simulink model "PFM"  (R2024a)
settings: Solver=ode15s  StartTime=0.0  StopTime=0.5  FixedStep=1e-8  RelTol=1e-5
values from neighbouring files (symbols this model uses):
  Cd = 33e-6    (= 3.3e-05)    [Results.m]
  Co = 200e-6    (= 0.0002)    [Results.m]
  Cpv = 100e-6    (= 0.0001)    [Results.m]
  Cr = 3e-6    (= 3e-06)    [Results.m]
  I1 = data.I1(N)    [Results.m]
  I2 = data.I2(N)    [Results.m]
  I3 = data.I3(N)    [Results.m]
  IR1 = Irradiance1    [Results.m]
  IR2 = Irradiance2    [Results.m]
  IR3 = Irradiance3    [Results.m]
  Lm = 8e-6    (= 8e-06)    [Results.m]
  Lr = 1e-6    (= 1e-06)    [Results.m]
  N = 3.5    [Results.m]
  Pactual = [data.P1(N) data.P2(N) data.P3(N)]    [Results.m]
  Rleak = 1    [Results.m]
  T = data.Temperature(N)    [Results.m]
  Vactual = [data.VP1(N) data.VP2(N) data.VP3(N)]    [Results.m]
  Vout = 120    [Results.m]
libraries: spsDiodeLib x8, spsParallelRLCBranchLib x7, spsCurrentMeasurementLib x7, spsMosfetLib x5, spsSeriesRLCBranchLib x3, spsPVArrayLib x3, spsVoltageMeasurementLib x3, spsOnDelayLib x2, spsLinearTransformerLib x1, spsDCVoltageSourceLib x1, spspowerguiLib x1
settings Model: Creator=user  LastModifiedBy=Donald
settings OptimizationCC: ZeroExternalMemoryAtStartup=off  ZeroInternalMemoryAtStartup=off
settings SFSimCC: SimTargetLang=C++
settings RTWCC: Toolchain=Microsoft Visual C++ 2017 v15.0 | CMake/nmake (64-bit Windows)  BuildConfiguration=Release  TargetLang=C++
settings GRTTargetCC: TargetLangStandard=C++11 (ISO)  CodeInterfacePackaging=C++ class

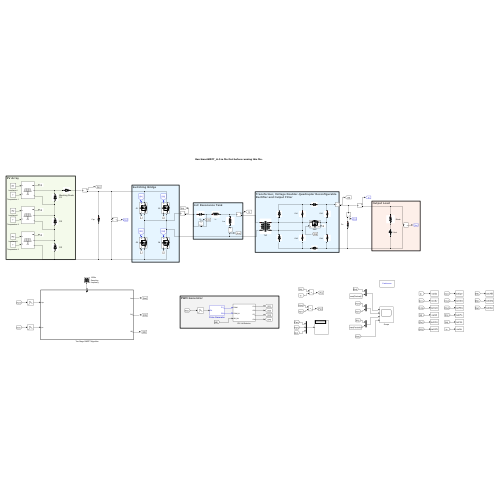
[thumbnail: Simulink's stored preview of the top-level diagram]
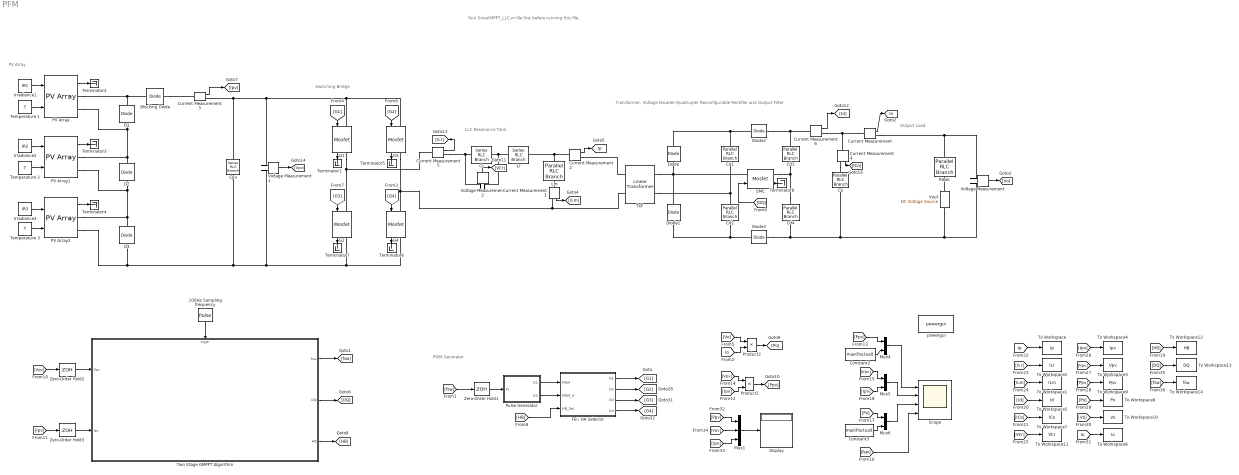
== system PFM ==
  note: LLC Resonance Tank
  note: PWM Generator
  note: PV Array
  note: Run SmartMPPT_LLC.m file first before running this file.
  note: Switching Bridge
  note: Output Load
  note: Transformer, Voltage Doubler-Quadrupler Reconfigurable
      | Rectifier and Output Filter
  100Hz Sampling frequency : DiscretePulseGenerator  PulseType=Time based  Period=1/100  PulseWidth=50
  Blocking Diode : spsDiodeLib/Diode  Ron=0.001  Lon=0  Vf=0.7  IC=0  UseSnubber=off  Rs=1e5*inf  Cs=inf  Measurements=off
  Cd{1..4} (4 alike) : spsParallelRLCBranchLib/Parallel RLC Branch  LConnTagsString=a  RConnTagsString=__new0  BranchType=C  Resistance=1  Inductance=1e-3  SetiL0=off  InitialCurrent=0  Capacitance=Cd  Setx0=off  InitialVoltage=0  Measurements=None
  Co : spsParallelRLCBranchLib/Parallel RLC Branch  LConnTagsString=a  RConnTagsString=__new0  BranchType=C  Resistance=1  Inductance=1e-3  SetiL0=off  InitialCurrent=0  Capacitance=Co  Setx0=off  InitialVoltage=0  Measurements=None
  Constant2 : Constant  Value=max(Pactual)
  Constant3 : Constant  Value=max(Pactual)
  Cpv : spsSeriesRLCBranchLib/Series RLC Branch  LConnTagsString=__new0  RConnTagsString=__new0  BranchType=C  Resistance=1  Inductance=1e-3  SetiL0=off  InitialCurrent=0  Capacitance=Cpv  Setx0=on  InitialVoltage=0  Measurements=None
  Cr : spsSeriesRLCBranchLib/Series RLC Branch  LConnTagsString=__new0  RConnTagsString=__new0  BranchType=C  Resistance=1  Inductance=1e-3  SetiL0=off  InitialCurrent=0  Capacitance=Cr  Setx0=off  InitialVoltage=0  Measurements=None
  Current Measurement{,1..6} (7 alike) : spsCurrentMeasurementLib/Current Measurement  PhasorSimulation=off  OutputType=Complex  PSBequivalent=0
  D1 : spsDiodeLib/Diode  Ron=0.001  Lon=0  Vf=0.7  IC=0  UseSnubber=off  Rs=1e5*inf  Cs=inf  Measurements=off
  D2 : spsDiodeLib/Diode  Ron=0.001  Lon=0  Vf=0.7  IC=0  UseSnubber=off  Rs=1e5*inf  Cs=inf  Measurements=off
  D3 : spsDiodeLib/Diode  Ron=0.001  Lon=0  Vf=0.7  IC=0  UseSnubber=off  Rs=1e5*inf  Cs=inf  Measurements=off
  Diode{,1..3} (4 alike) : spsDiodeLib/Diode  Ron=1e-3  Lon=0  Vf=0  IC=0  UseSnubber=0  Rs=inf  Cs=0  Measurements=off
  Display : Display
  FB / HA Selector : Subsystem
  G1 : spsMosfetLib/Mosfet  Ron=1e-3  Lon=0  Rd=1e-3  Vfd=0  IC=0  Rs=10e3  Cs=0.1e-6  Measurements=on
  G2 : spsMosfetLib/Mosfet  Ron=1e-3  Lon=0  Rd=1e-3  Vfd=0  IC=0  Rs=10e3  Cs=0.1e-6  Measurements=on
  G3 : spsMosfetLib/Mosfet  Ron=1e-3  Lon=0  Rd=1e-3  Vfd=0  IC=0  Rs=10e3  Cs=0  Measurements=on
  G4 : spsMosfetLib/Mosfet  Ron=1e-3  Lon=0  Rd=1e-3  Vfd=0  IC=0  Rs=10e3  Cs=0.1e-6  Measurements=on
  Irradiance1 : Constant  Value=IR1
  Irradiance2 : Constant  Value=IR2
  Irradiance3 : Constant  Value=IR3
  Lm : spsParallelRLCBranchLib/Parallel RLC Branch  LConnTagsString=a  RConnTagsString=__new0  BranchType=L  Resistance=1  Inductance=Lm  SetiL0=off  InitialCurrent=0  Capacitance=1e-6  Setx0=off  InitialVoltage=0  Measurements=None
  Lr : spsSeriesRLCBranchLib/Series RLC Branch  LConnTagsString=__new0  RConnTagsString=__new0  BranchType=L  Resistance=1  Inductance=Lr  SetiL0=off  InitialCurrent=0  Capacitance=2.91e-6  Setx0=off  InitialVoltage=0  Measurements=None
  Mux1 : Mux  Inputs=3
  Mux4 : Mux  Inputs=2
  Mux5 : Mux  Inputs=2
  Mux6 : Mux  Inputs=2
  PV Array : spsPVArrayLib/PV Array  Npar=1  Nser=1  PlotType=array @ 25 deg.C & specified irradiances  S_vec="[ 1000  600  100 ]"  Temp_C_vec="[ 45 25  ]"  ModuleName=User-defined  PlotWhenSelected=off  Pm=83.2824  Ncell=60/3  Voc=37.92*20/60  Isc=8.62  Vm=30.96*20/60  Im=8.07  beta_Voc_pc=-0.36099  alpha_Isc_pc=0.06371  beta_Voc=-0.045629  alpha_Isc=0.0054918  IL=8.6465  I0=3.0335e-10  nI=1.0227  Rsh=76.0432  Rs=0.09434  RobustModel=off  RobustCellTemperature=313.3991  BAL=on  Tc=1e-6  Tfilter=5e-5
  PV Array1 : spsPVArrayLib/PV Array  Npar=1  Nser=1  PlotType=array @ 25 deg.C & specified irradiances  S_vec="[ 1000  600  100 ]"  Temp_C_vec="[ 45 25  ]"  ModuleName=User-defined  PlotWhenSelected=off  Pm=83.2824  Ncell=60/3  Voc=37.92*20/60  Isc=8.62  Vm=30.96*20/60  Im=8.07  beta_Voc_pc=-0.36099  alpha_Isc_pc=0.06371  beta_Voc=-0.045629  alpha_Isc=0.0054918  IL=8.6465  I0=3.0335e-10  nI=1.0227  Rsh=76.0432  Rs=0.09434  RobustModel=off  RobustCellTemperature=313.3991  BAL=on  Tc=1e-6  Tfilter=5e-5
  PV Array2 : spsPVArrayLib/PV Array  Npar=1  Nser=1  PlotType=array @ 25 deg.C & specified irradiances  S_vec="[ 1000  600  100 ]"  Temp_C_vec="[ 45 25  ]"  ModuleName=User-defined  PlotWhenSelected=off  Pm=83.2824  Ncell=60/3  Voc=37.92*20/60  Isc=8.62  Vm=30.96*20/60  Im=8.07  beta_Voc_pc=-0.36099  alpha_Isc_pc=0.06371  beta_Voc=-0.045629  alpha_Isc=0.0054918  IL=8.6465  I0=3.0335e-10  nI=1.0227  Rsh=76.0432  Rs=0.09434  RobustModel=off  RobustCellTemperature=313.3991  BAL=on  Tc=1e-6  Tfilter=5e-5
  Product1 : Product
  Product2 : Product
  Pulse Generator : Subsystem
  Rleak : spsParallelRLCBranchLib/Parallel RLC Branch  LConnTagsString=a  RConnTagsString=__new0  BranchType=R  Resistance=Rleak  Inductance=1.193e-05  SetiL0=off  InitialCurrent=0  Capacitance=1e-6  Setx0=off  InitialVoltage=0  Measurements=None
  SMC : spsMosfetLib/Mosfet  Ron=1e-3  Lon=0  Rd=1e-3  Vfd=0  IC=0  Rs=10e3  Cs=0  Measurements=on
  Scope : Scope  NumInputPorts=4
  TXF : spsLinearTransformerLib/Linear Transformer  UNITS=pu  NominalPower=[1000 100e3 ]  winding1=[1 0 0]  winding2=[N 0 0]  ThreeWindings=off  winding3=[ 315e3 0.002 0.08 ]  RmLm=[ 1e6 inf ]  Measurements=None  DataType=off
  Temperature 1 : Constant  Value=T
  Temperature 2 : Constant  Value=T
  Temperature 3 : Constant  Value=T
  Terminator{1..8} (8 alike) : Terminator
  To Workspace : ToWorkspace  VariableName=Ip  SaveFormat=Timeseries  SampleTime=-1
  To Workspace1 : ToWorkspace  VariableName=ILm  SaveFormat=Timeseries  SampleTime=-1
  To Workspace10 : ToWorkspace  VariableName=Vo  SaveFormat=Timeseries  SampleTime=-1
  To Workspace11 : ToWorkspace  VariableName=VCr  SaveFormat=Timeseries  SampleTime=-1
  To Workspace12 : ToWorkspace  VariableName=HB  SaveFormat=Timeseries  SampleTime=-1
  To Workspace13 : ToWorkspace  VariableName=DQ  SaveFormat=Timeseries  SampleTime=-1
  To Workspace14 : ToWorkspace  VariableName=fsw  SaveFormat=Timeseries  SampleTime=-1
  To Workspace2 : ToWorkspace  VariableName=ILr  SaveFormat=Timeseries  SampleTime=-1
  To Workspace3 : ToWorkspace  VariableName=Vpv  SaveFormat=Timeseries  SampleTime=-1
  To Workspace4 : ToWorkspace  VariableName=Ipv  SaveFormat=Timeseries  SampleTime=-1
  To Workspace5 : ToWorkspace  VariableName=Id  SaveFormat=Timeseries  SampleTime=-1
  To Workspace6 : ToWorkspace  VariableName=Io  SaveFormat=Timeseries  SampleTime=-1
  To Workspace7 : ToWorkspace  VariableName=ICo  SaveFormat=Timeseries  SampleTime=-1
  To Workspace8 : ToWorkspace  VariableName=Po  SaveFormat=Timeseries  SampleTime=-1
  To Workspace9 : ToWorkspace  VariableName=Ppv  SaveFormat=Timeseries  SampleTime=-1
  Two Stage GMPPT Algorithm : Subsystem  TreatAsAtomicUnit=on
  Voltage Measurement : spsVoltageMeasurementLib/Voltage Measurement  PhasorSimulation=off  OutputType=Complex  PSBequivalent=0
  Voltage Measurement1 : spsVoltageMeasurementLib/Voltage Measurement  PhasorSimulation=off  OutputType=Complex  PSBequivalent=0
  Voltage Measurement2 : spsVoltageMeasurementLib/Voltage Measurement  PhasorSimulation=off  OutputType=Complex  PSBequivalent=0
  Vout : spsDCVoltageSourceLib/DC Voltage Source  Amplitude=Vout  Measurements=None
  Zero-Order Hold1 : ZeroOrderHold  SampleTime=1/100e3
  Zero-Order Hold2 : ZeroOrderHold  SampleTime=1/100e3
  Zero-Order Hold3 : ZeroOrderHold  SampleTime=1/100e3
  powergui : spspowerguiLib/powergui  Priority=1  SimulationMode=Continuous  SampleTime=1e-8  frequency=60  Iterations=50  frequencyindice=0  Pbase=100e6  ErrMax=1e-4  UnitsV=kV  UnitsW=MW  buscounter=0  FunctionMessages=off  echomessages=off  EnableUseOfTLC=off  CurrentSourceSwitches=off  DisableSnubberDevices=off  DisableRonSwitches=off  DisableVfSwitches=off  DisplayEquations=off  AutomaticDiscreteSolvers=off  SolverType=Tustin/Backward Euler (TBE)  Interpol=off  ExternalGateDelay=off  methode=off  Ts=100  x0status=blocks  SPID=on  SwTol=0  HookPort=off  NonlinearTolerance=1e-4  nMaxIteration=100  ContinueOnMaxIteration=off  RestoreLinks=warning  ResistiveCurrentMeasurement=off  Frange=[0:2:500]  Ylog=off  Xlog=on  ShowGrid=off  save=off  variable=ZData  structure=0  ZoomFFT=off  StartTime=0.0  cycles=1  DisplayStyle=1  fundamental=60  FreqAxis=off  MaxFrequency=1000  frequencyindicesteady=1  RmsSteady=1  display=off
  tag scope: Io=global, Ip=global
  wires:
  Current Measurement5/1 -> [ILr]
  Current Measurement1/1 -> [ILm]
  Current Measurement2/1 -> [Ip]
  [G4] -> G4/1
  [G1] -> G1/1
  [G3] -> G2/1
  [G2] -> G3/1
  Irradiance1/1 -> PV Array/1
  Irradiance2/1 -> PV Array1/1
  Irradiance3/1 -> PV Array2/1
  Temperature 2/1 -> PV Array1/2
  PV Array/1 -> Terminator2/1
  PV Array2/1 -> Terminator4/1
  Temperature 3/1 -> PV Array2/2
  PV Array1/1 -> Terminator3/1
  Temperature 1/1 -> PV Array/2
  Zero-Order Hold1/1 -> Pulse Generator/1(Fs)
  G1/1 -> Terminator1/1
  G3/1 -> Terminator5/1
  G4/1 -> Terminator6/1
  G2/1 -> Terminator7/1
  [DQ] -> SMC/1
  Current Measurement6/1 -> [Id]
  SMC/1 -> Terminator8/1
  Current Measurement4/1 -> [ICo]
  FB / HA Selector/3(G3) -> [G3]
  FB / HA Selector/2(G2) -> [G2]
  Pulse Generator/2(G2) -> FB / HA Selector/2(PWM_N)
  FB / HA Selector/4(G4) -> [G4]
  FB / HA Selector/1(G1) -> [G1]
  Pulse Generator/1(G1) -> FB / HA Selector/1(PWM)
  [fsw] -> Zero-Order Hold1/1
  100Hz Sampling frequency/1 -> Two Stage GMPPT Algorithm/Trigger
  Zero-Order Hold2/1 -> Two Stage GMPPT Algorithm/1(Vpv)
  Zero-Order Hold3/1 -> Two Stage GMPPT Algorithm/2(Ipv)
  Two Stage GMPPT Algorithm/1(fsw) -> [fsw]
  Two Stage GMPPT Algorithm/3(HB) -> [HB]
  Two Stage GMPPT Algorithm/2(DQ) -> [DQ]
  [HB] -> FB / HA Selector/3(HB_Sel)
  [Vpv] -> Zero-Order Hold2/1
  [Ipv] -> Zero-Order Hold3/1
  Current Measurement3/1 -> [Ipv]
  Voltage Measurement1/1 -> [Vpv]
  Voltage Measurement/1 -> [Vo]
  Current Measurement/1 -> [Io]
  Voltage Measurement2/1 -> [VCr]
  [Ppv] -> Mux1/1
  [Vo] -> To Workspace10/1
  [Po] -> To Workspace8/1
  [Ppv] -> To Workspace9/1
  [Vpv] -> To Workspace3/1
  [ICo] -> To Workspace7/1
  [Vo] -> Product2/1
  [Ipv] -> To Workspace4/1
  [Io] -> To Workspace6/1
  [Id] -> To Workspace5/1
  [VCr] -> To Workspace11/1
  [Ip] -> To Workspace/1
  [fsw] -> Scope/4
  Mux1/1 -> Display/1
  Product1/1 -> [Ppv]
  [Io] -> Product2/2
  Product2/1 -> [Po]
  [ILm] -> To Workspace1/1
  [Po] -> Mux6/1
  Constant2/1 -> Mux4/2
  Constant3/1 -> Mux6/2
  [Vpv] -> Product1/1
  Mux4/1 -> Scope/1
  [Ipv] -> Product1/2
  Mux6/1 -> Scope/3
  [Ipv] -> Mux1/3
  [Ipv] -> Mux5/2
  Mux5/1 -> Scope/2
  [Vpv] -> Mux1/2
  [Vpv] -> Mux5/1
  [ILr] -> To Workspace2/1
  [Ppv] -> Mux4/1
  [DQ] -> To Workspace13/1
  [HB] -> To Workspace12/1
  [fsw] -> To Workspace14/1
  connections:
  Lm/LConn1 -- Current Measurement2/LConn1 -- Lr/RConn1
  Lr/LConn1 -- Voltage Measurement2/LConn2 -- Cr/RConn1
  Voltage Measurement2/LConn1 -- Current Measurement5/RConn1 -- Cr/LConn1
  Lm/RConn1 -- Current Measurement1/LConn1
  TXF/LConn1 -- Current Measurement2/RConn1
  G3/RConn1 -- G4/LConn1 -- TXF/LConn2 -- Current Measurement1/RConn1
  G2/LConn1 -- G1/RConn1 -- Current Measurement5/LConn1
  G3/LConn1 -- Current Measurement3/RConn1 -- Cpv/LConn1 -- Voltage Measurement1/LConn1 -- G1/LConn1
  G2/RConn1 -- G4/RConn1 -- Voltage Measurement1/LConn2 -- Cpv/RConn1 -- D3/LConn1 -- PV Array2/RConn2
  PV Array1/RConn1 -- D2/RConn1 -- PV Array/RConn2 -- D1/LConn1
  PV Array1/RConn2 -- PV Array2/RConn1 -- D3/RConn1 -- D2/LConn1
  D1/RConn1 -- PV Array/RConn1 -- Blocking Diode/LConn1
  Blocking Diode/RConn1 -- Current Measurement3/LConn1
  Diode/RConn1 -- Diode2/LConn1 -- Cd1/LConn1
  Diode2/RConn1 -- Cd3/LConn1 -- Current Measurement6/LConn1
  Cd2/LConn1 -- TXF/RConn2 -- Cd1/RConn1
  Cd4/LConn1 -- Cd3/RConn1 -- SMC/RConn1
  Current Measurement/LConn1 -- Current Measurement4/LConn1 -- Current Measurement6/RConn1
  Diode1/RConn1 -- TXF/RConn1 -- SMC/LConn1 -- Diode/LConn1
  Voltage Measurement/LConn1 -- Rleak/LConn1 -- Current Measurement/RConn1
  Vout/LConn1 -- Voltage Measurement/LConn2 -- Co/RConn1 -- Cd4/RConn1 -- Diode3/LConn1
  Diode1/LConn1 -- Diode3/RConn1 -- Cd2/RConn1
  Vout/RConn1 -- Rleak/RConn1
  Current Measurement4/RConn1 -- Co/LConn1

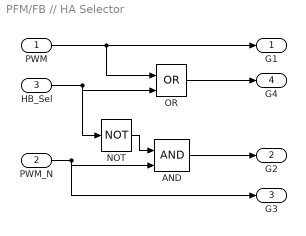
== system PFM/FB // HA Selector ==
  PWM : Inport
  PWM_N : Inport  Port=2
  HB_Sel : Inport  Port=3
  AND : Logic  IconShape=distinctive  AllPortsSameDT=off  OutDataTypeStr=boolean
  NOT : Logic  Operator=NOT  IconShape=distinctive  AllPortsSameDT=off  OutDataTypeStr=boolean
  OR : Logic  Operator=OR  IconShape=distinctive  AllPortsSameDT=off  OutDataTypeStr=boolean
  G1 : Outport
  G2 : Outport  Port=2
  G3 : Outport  Port=3
  G4 : Outport  Port=4
  wires:
  OR/1 -> G4/1
  PWM/1 -> OR/1, G1/1
  HB_Sel/1 -> NOT/1, OR/2
  PWM_N/1 -> AND/2, G3/1
  AND/1 -> G2/1
  NOT/1 -> AND/1

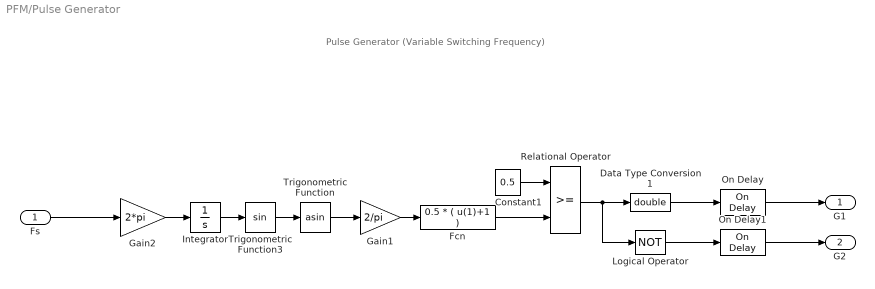
== system PFM/Pulse Generator ==
  note: Pulse Generator
      | (Variable Switching Frequency)
  Fs : Inport
  Constant1 : Constant  Value=0.5
  Data Type Conversion1 : DataTypeConversion  OutDataTypeStr=double  SaturateOnIntegerOverflow=off  RndMeth=Floor
  Fcn : Fcn  Expr=0.5 * ( u(1)+1 )
  Gain1 : Gain  Gain=2/pi  SaturateOnIntegerOverflow=on  OutDataTypeStr=Inherit: Same as input  ParamDataTypeStr=Inherit: Same as input
  Gain2 : Gain  Gain=2*pi  SaturateOnIntegerOverflow=on  OutDataTypeStr=Inherit: Same as input  ParamDataTypeStr=Inherit: Same as input
  Integrator : Integrator
  Logical Operator : Logic  Operator=NOT  AllPortsSameDT=off  OutDataTypeStr=float('double')
  On Delay : spsOnDelayLib/On Delay  DelayType=On delay  delay=400e-9  ic=0  Ts=0
  On Delay1 : spsOnDelayLib/On Delay  DelayType=On delay  delay=400e-9  ic=0  Ts=0
  Relational Operator : RelationalOperator  OutDataTypeStr=boolean  InputSameDT=off
  Trigonometric Function : Trigonometry  Operator=asin
  Trigonometric Function3 : Trigonometry
  G1 : Outport  VectorParamsAs1DForOutWhenUnconnected=off
  G2 : Outport  Port=2  VectorParamsAs1DForOutWhenUnconnected=off
  wires:
  Trigonometric Function3/1 -> Trigonometric Function/1
  Gain1/1 -> Fcn/1
  Trigonometric Function/1 -> Gain1/1
  Integrator/1 -> Trigonometric Function3/1
  Constant1/1 -> Relational Operator/1
  Relational Operator/1 -> Data Type Conversion1/1, Logical Operator/1
  Fcn/1 -> Relational Operator/2
  Logical Operator/1 -> On Delay1/1
  Data Type Conversion1/1 -> On Delay/1
  Gain2/1 -> Integrator/1
  Fs/1 -> Gain2/1
  On Delay/1 -> G1/1
  On Delay1/1 -> G2/1

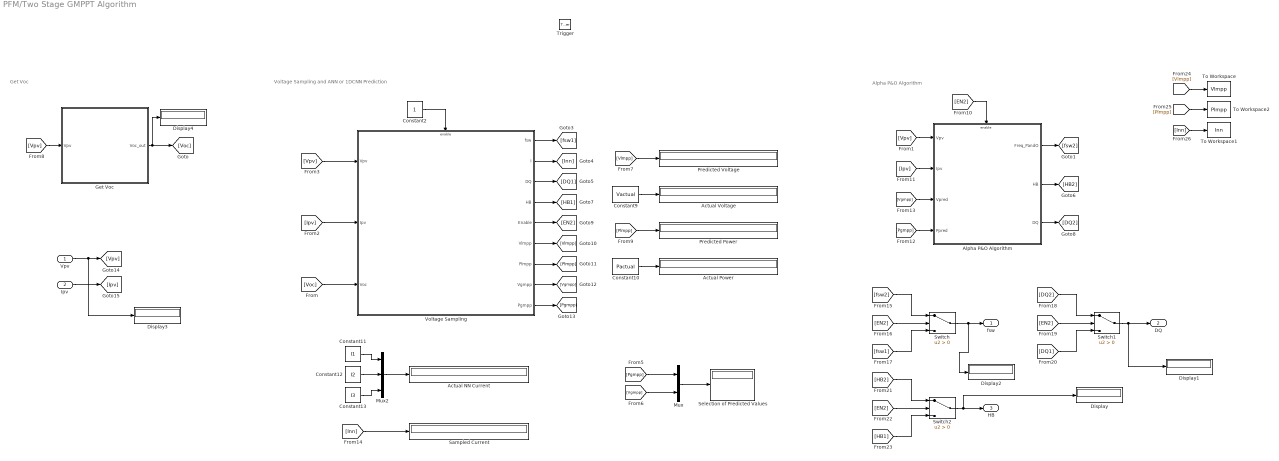
== system PFM/Two Stage GMPPT Algorithm ==
  note: Voltage Sampling and ANN or 1DCNN Prediction
  note: Alpha P&O Algorithm
  note: Get Voc
  Vpv : Inport
  Ipv : Inport  Port=2
  Trigger : TriggerPort  VariantControl=(inherit)  InitialTriggerSignalState=positive  PortDimensions=1
  Actual NN Current : Display
  Actual Power : Display
  Actual Voltage : Display
  Alpha P&O Algorithm : Subsystem  TreatAsAtomicUnit=on
  Constant10 : Constant  Value=Pactual
  Constant11 : Constant  Value=I1
  Constant12 : Constant  Value=I2
  Constant13 : Constant  Value=I3
  Constant2 : Constant
  Constant9 : Constant  Value=Vactual
  Display{,1..4} (5 alike) : Display
  Get Voc : MATLAB Function  TreatAsAtomicUnit=on
  Mux : Mux  Inputs=2
  Mux2 : Mux  Inputs=3
  Predicted Power : Display
  Predicted Voltage : Display
  Sampled Current : Display
  Selection of Predicted Values : Display
  Switch : Switch  Criteria=u2 > Threshold  SaturateOnIntegerOverflow=off  InputSameDT=off
  Switch1 : Switch  Criteria=u2 > Threshold  SaturateOnIntegerOverflow=off  InputSameDT=off
  Switch2 : Switch  Criteria=u2 > Threshold  SaturateOnIntegerOverflow=off  InputSameDT=off
  To Workspace : ToWorkspace  VariableName=Vlmpp  SaveFormat=Timeseries  SampleTime=-1
  To Workspace1 : ToWorkspace  VariableName=Inn  SaveFormat=Timeseries  SampleTime=-1
  To Workspace2 : ToWorkspace  VariableName=Plmpp  SaveFormat=Timeseries  SampleTime=-1
  Voltage Sampling : Subsystem  TreatAsAtomicUnit=on
  fsw : Outport
  DQ : Outport  Port=2
  HB : Outport  Port=3
  wires:
  Mux2/1 -> Actual NN Current/1
  [Pgmpp] -> Mux/1
  [EN2] -> Alpha P&O Algorithm/Enable
  Constant12/1 -> Mux2/2
  Alpha P&O Algorithm/1(Freq_PandO) -> [fsw2]
  Constant13/1 -> Mux2/3
  Constant11/1 -> Mux2/1
  Mux/1 -> Selection of Predicted Values/1
  [Voc] -> Voltage Sampling/3(Voc)
  [Vpv] -> Voltage Sampling/1(Vpv)
  [Ipv] -> Voltage Sampling/2(Ipv)
  Voltage Sampling/1(fsw) -> [fsw1]
  Voltage Sampling/2(I) -> [Inn]
  Voltage Sampling/9(Pgmpp) -> [Pgmpp]
  Voltage Sampling/8(Vgmpp) -> [Vgmpp]
  Voltage Sampling/7(Plmpp) -> [Plmpp]
  Voltage Sampling/6(Vlmpp) -> [Vlmpp]
  Voltage Sampling/5(Enable) -> [EN2]
  Voltage Sampling/4(HB) -> [HB1]
  Voltage Sampling/3(DQ) -> [DQ1]
  [Vgmpp] -> Mux/2
  Constant10/1 -> Actual Power/1
  [Plmpp] -> Predicted Power/1
  Constant9/1 -> Actual Voltage/1
  [Vlmpp] -> Predicted Voltage/1
  Alpha P&O Algorithm/2(HB) -> [HB2]
  Alpha P&O Algorithm/3(DQ) -> [DQ2]
  [Vpv] -> Alpha P&O Algorithm/1(Vpv)
  [Ipv] -> Alpha P&O Algorithm/2(Ipv)
  [Vgmpp] -> Alpha P&O Algorithm/3(Vpred)
  [Pgmpp] -> Alpha P&O Algorithm/4(Ppred)
  Vpv/1 -> Display3/1, [Vpv]
  Ipv/1 -> [Ipv]
  [Inn] -> Sampled Current/1
  [EN2] -> Switch/2
  [fsw2] -> Switch/1
  [fsw1] -> Switch/3
  Switch/1 -> Display2/1, fsw/1
  [DQ1] -> Switch1/3
  [DQ2] -> Switch1/1
  [EN2] -> Switch1/2
  Switch1/1 -> Display1/1, DQ/1
  Switch2/1 -> Display/1, HB/1
  [HB1] -> Switch2/3
  [HB2] -> Switch2/1
  [EN2] -> Switch2/2
  [Vpv] -> Get Voc/1(Vpv)
  Get Voc/1(Voc_out) -> [Voc], Display4/1
  Constant2/1 -> Voltage Sampling/Enable
  [Plmpp] -> To Workspace2/1
  [Inn] -> To Workspace1/1
  [Vlmpp] -> To Workspace/1

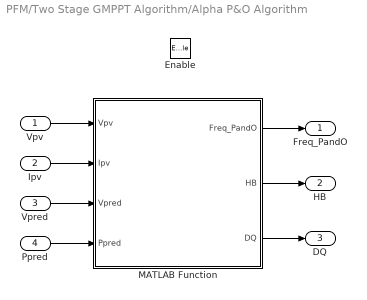
== system PFM/Two Stage GMPPT Algorithm/Alpha P&O Algorithm ==
  Vpv : Inport
  Ipv : Inport  Port=2
  Vpred : Inport  Port=3
  Ppred : Inport  Port=4
  Enable : EnablePort
  MATLAB Function : MATLAB Function  TreatAsAtomicUnit=on
  Freq_PandO : Outport
  HB : Outport  Port=2
  DQ : Outport  Port=3
  wires:
  Ppred/1 -> MATLAB Function/4(Ppred)
  Vpv/1 -> MATLAB Function/1(Vpv)
  MATLAB Function/3(DQ) -> DQ/1
  Vpred/1 -> MATLAB Function/3(Vpred)
  MATLAB Function/1(Freq_PandO) -> Freq_PandO/1
  MATLAB Function/2(HB) -> HB/1
  Ipv/1 -> MATLAB Function/2(Ipv)

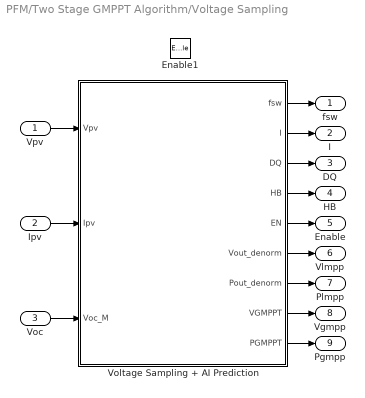
== system PFM/Two Stage GMPPT Algorithm/Voltage Sampling ==
  Vpv : Inport
  Ipv : Inport  Port=2
  Voc : Inport  Port=3
  Enable1 : EnablePort
  Voltage Sampling + AI Prediction : MATLAB Function  TreatAsAtomicUnit=on
  fsw : Outport
  I : Outport  Port=2
  DQ : Outport  Port=3
  HB : Outport  Port=4
  Enable : Outport  Port=5
  Vlmpp : Outport  Port=6
  Plmpp : Outport  Port=7
  Vgmpp : Outport  Port=8
  Pgmpp : Outport  Port=9
  wires:
  Voltage Sampling + AI Prediction/4(HB) -> HB/1
  Voltage Sampling + AI Prediction/3(DQ) -> DQ/1
  Voltage Sampling + AI Prediction/5(EN) -> Enable/1
  Voltage Sampling + AI Prediction/1(fsw) -> fsw/1
  Voltage Sampling + AI Prediction/2(I) -> I/1
  Vpv/1 -> Voltage Sampling + AI Prediction/1(Vpv)
  Ipv/1 -> Voltage Sampling + AI Prediction/2(Ipv)
  Voltage Sampling + AI Prediction/6(Vout_denorm) -> Vlmpp/1
  Voltage Sampling + AI Prediction/7(Pout_denorm) -> Plmpp/1
  Voltage Sampling + AI Prediction/8(VGMPPT) -> Vgmpp/1
  Voltage Sampling + AI Prediction/9(PGMPPT) -> Pgmpp/1
  Voc/1 -> Voltage Sampling + AI Prediction/3(Voc_M)

== matlab function PFM/Two Stage GMPPT Algorithm/Get Voc ==
  data: Vpv input; Voc_out output
function Voc_out  = VocSample(Vpv)
    % Store measurement for the current frequency.
    persistent Voc;
    
    % Initialize persistent variables only once
    if isempty(Voc)
        Voc = Vpv;
    end
    
    if Vpv > Voc
        Voc = Vpv;
    end
    Voc_out = Voc;
end

== matlab function PFM/Two Stage GMPPT Algorithm/Alpha P&O Algorithm/MATLAB Function ==
  data: Vpv input; Freq_PandO output; Ipv input; Vpred input; Ppred input; HB output; DQ output
function [Freq_PandO, HB, DQ] = PandO(Vpv, Ipv, Vpred, Ppred)
    % Constants.
    delta_freq = 2e3;
    
    % Current power.
    Ppv = Vpv * Ipv;
    
    % Persistent variables to retain values between function calls.
    persistent Vold Pold Fcalc HB_old DQ_old;

    % Initialize persistent variables on the first function call.
    if isempty(Fcalc)
        Vold = Vpred;        % Store the initial predicted voltage for ANN.
        Pold = Ppred;        % Store the initial predicted power for ANN.
        Fcalc = 0;
        if Vpred > 21
            DQ_old = 0;
            HB_old = 1;
            Gain = 120/Vpred /3.5/2*2;
            Fcalc = FMIM(Ppred, Gain);
        elseif Vpred > 11
            DQ_old = 0;
            HB_old = 0;
            Gain = 120/Vpred /3.5/2;
            Fcalc = FMIM(Ppred, Gain);
        else
            DQ_old = 1;
            HB_old = 0;
            Gain = 120/Vpred /3.5/2/2;
            Fcalc = FMIM(Ppred, Gain);
        end
        
        % Output initial voltage on the first call.
        Freq_PandO = Fcalc; 
        HB = HB_old;
        DQ = DQ_old;
        return;            % Exit early during initialization.
    end
    
    % Try use sigmoid.
    factor = 1/(1+exp(-abs(Ppv - Pold)));

    % P&O algorithm logic.
    if abs(Ppv - Pold) < 0.01  % Threshold to account for floating-point precision.
        % If power has not significantly changed, retain the previous
        % calculated frequency.
        Freq_PandO = Fcalc;
        HB = HB_old;
        DQ = DQ_old;
    else
        % Decide voltage adjustment based on power and voltage changes.
        if (Ppv - Pold) < 0
            % Power decreased
            if (Vpv - Vold) < 0
                Fcalc = Fcalc + delta_freq*factor; % Increase the voltage.
            else
                Fcalc = Fcalc - delta_freq*factor; % Decrease the voltage.
            end
        else
            % Power increased.
            if (Vpv - Vold) < 0
                Fcalc = Fcalc - delta_freq; % Decrease the voltage.
            else
                Fcalc = Fcalc + delta_freq; % Increase the voltage.
            end
        end
        
        % Update the output voltage after adjustment.
        Freq_PandO = Fcalc;
        HB = HB_old;
        DQ = DQ_old;
    end

    % Update the previous voltage and power for the next iteration.
    Vold = Vpv;
    Pold = Ppv;
end


function f0 = FMIM(P_assumed, Gain)
    % FMIM performs the initial switching frequency estimation based on
    % the FMIM method using an assumed power level.
    %
    % Inputs:
    %   Vref      - Reference voltage.
    %   P_assumed - Assumed power (W) (e.g., 50 or 100 W).
    %
    % Output:
    %   f0 - Estimated switching frequency.
    
    % LLC converter parameters.
    Cr = 3e-6;
    Lr = 1e-6;
    Lm = 8e-6;
    
    % Output voltage.
    Vout = 120;
    
    % Calculate load resistance assuming 100% efficiency.
    Rload = Vout^2 / P_assumed;
    % Transformer turns ratio.
    N = 1/5;
    % Effective AC resistance for full-bridge LLC converter.
    Rac = (8/pi^2) * (N^2) * (1/4) * Rload;
    
    % Define key parameters.
    K = Lm / Lr;
    Q = sqrt(Lr / Cr) / Rac;
    
    % Cubic equation's coefficients.
    a = 1;
    b = ((K^(-2)*(K+1)^2) - (2*Q^2) - (Gain^(-2))) / (Q^2);
    c = (Q^2 - (2*K^(-2) * (K + 1))) / (Q^2);
    d = (1 / (K * Q))^2;
    
    % Solve the cubic equation and take the square roots of the roots.
    fn_array = sqrt(roots([a b c d]));
    fn = max(real(fn_array));
    
    % Calculate resonance frequency.
    fr = 1 / (2 * pi * sqrt(Lr * Cr));
    
    % Estimated switching frequency.
    f0 = fn * fr;
end

== matlab function PFM/Two Stage GMPPT Algorithm/Voltage Sampling/Voltage Sampling + AI Prediction ==
  data: Vpv input; Ipv input; fsw output; I output; DQ output; HB output; EN output; Vout_denorm output; Pout_denorm output; VGMPPT output; PGMPPT output; Voc_M input
function [fsw, I, DQ, HB, EN, Vout_denorm, Pout_denorm, VGMPPT, PGMPPT] = SearchVref(Vpv, Ipv, Voc_M)
    % Store measurement for the current frequency.
    persistent NSample Vref targetVal Inn InnFlag fold DQ_Sel HB_EN ENC Vout_denorm_old Pout_denorm_old VGMPPT_old PGMPPT_old;
    
    if isempty(fold)
        % /////////////////////////////////////////////////////////////
        % Voltage scanning param.
        % /////////////////////////////////////////////////////////////
        NSample = 0;  
        Vref = [0.4*12.64, 0.4+12.64, 0.4+2*12.64];
        targetVal = Vref(1);
        Inn = zeros(1, 3);
        I = Inn;
        InnFlag = zeros(1,3);

        [fold, HB_EN, DQ_Sel] = initializeSearchVref(targetVal, 35);
        DQ = DQ_Sel;
        HB = HB_EN;

        % Copy frequency to persistence and 48kHz < fsw < 250kHz.
        fold = max(45e3, fold);
        fold = min(250e3, fold);
        fsw = fold;
        % /////////////////////////////////////////////////////////////
        
        % Done ANN and voltage sampling ?
        ENC = 0;
        EN = ENC;
        
        % ANN param.
        Vout_denorm_old = [0 0 0];
        Pout_denorm_old = [0 0 0];
        VGMPPT_old = 0;
        PGMPPT_old = 0;
        Vout_denorm = Vout_denorm_old;
        Pout_denorm = Pout_denorm_old;
        VGMPPT = VGMPPT_old;
        PGMPPT = PGMPPT_old;
        return;
    end
    
    
    if ENC == 0
        NSample = NSample + 1;
        
        % Check each target voltage (Threshold from Jerome).
        for i = 1:3
            if (abs(Vref(i) - Vpv) < 2.1) && ~InnFlag(i)
                Inn(i) = Ipv;
                InnFlag(i) = 1;
                if InnFlag(1) == 0
                    targetVal = Vref(1);
                    [fold, HB_EN, DQ_Sel] = initializeSearchVref(targetVal, 35);
                elseif InnFlag(2) == 0
                    targetVal = Vref(2);
                    [fold, HB_EN, DQ_Sel] = initializeSearchVref(targetVal, 70);
                elseif InnFlag(3) == 0
                    targetVal = Vref(3);
                    [fold, HB_EN, DQ_Sel] = initializeSearchVref(targetVal, 60);
                else
                    ENC = 1;
                    [Vout_denorm_old, Pout_denorm_old, VGMPPT_old, PGMPPT_old] = tflite_predict(double(Inn(1)), double(Inn(2)), double(Inn(3)), double(Voc_M));

                end
                DQ = DQ_Sel;
                HB = HB_EN;
                EN = ENC;
                fsw = fold;
                I = Inn;
                
                Vout_denorm = Vout_denorm_old;
                Pout_denorm = Pout_denorm_old;
                VGMPPT = VGMPPT_old;
                PGMPPT = PGMPPT_old;

                disp('--/////////////////////');
                disp(Vref);
                disp(Vpv);
                disp(fold);
                disp(Inn);
                disp(InnFlag);
                disp(NSample);
                disp('--/////////////////////');
                return;
            end
        end

        fold = sliding_surface_control(targetVal, Vpv, fold);
         
        % Constrain fsw to a valid range (40kHz to infinity Hz).
        fold = max(45e3, fold);
        fold = min(250e3, fold);
        
        DQ = DQ_Sel;
        HB = HB_EN;
        ENC = 0;
        EN = ENC;
        fsw = fold;
        I = Inn;
        
        Vout_denorm = Vout_denorm_old;
        Pout_denorm = Pout_denorm_old;
        VGMPPT = VGMPPT_old;
        PGMPPT = PGMPPT_old;

        disp('/////////////////////');
        disp(Vref);
        disp(Vpv);
        disp(fold);
        disp(Inn);
        disp(InnFlag);
        disp(NSample);
        disp('/////////////////////');
    else
        DQ = DQ_Sel;
        HB = HB_EN;
        EN = ENC;
        fsw = fold;
        I = Inn;

        Vout_denorm = Vout_denorm_old;
        Pout_denorm = Pout_denorm_old;
        VGMPPT = VGMPPT_old;
        PGMPPT = PGMPPT_old;
    end
end


function [fsw, HB, DQ] = initializeSearchVref(Vref, P)
        Pass = P;
        if Vref > 21
            DQ_Sel = 0;
            HB_EN = 1;
            Gain = 120/Vref /3.5/2*2;
            fold = FMIM(Pass, Gain);
        elseif Vref > 11
            DQ_Sel = 0;
            HB_EN = 0;
            Gain = 120/Vref /3.5/2;
            fold = FMIM(Pass, Gain);
        else
            DQ_Sel = 1;
            HB_EN = 0;
            Gain = 120/Vref /3.5/2/2;
            fold = FMIM(Pass, Gain);
        end
    
        % Copy frequency to persistence and 48kHz < fsw < 250kHz.
        fold = max(45e3, fold);
        fold = min(250e3, fold);
        fsw = fold;
        
        HB = HB_EN;
        DQ = DQ_Sel;
end


function f0 = FMIM(P_assumed, Gain)
    % FMIM performs the initial switching frequency estimation based on
    % the FMIM method using an assumed power level.
    %
    % Inputs:
    %   Vref      - Reference voltage.
    %   P_assumed - Assumed power (W) (e.g., 50 or 100 W).
    %
    % Output:
    %   f0 - Estimated switching frequency.
    
    % LLC converter parameters.
    Cr = 3e-6;
    Lr = 1e-6;
    Lm = 8e-6;
    
    % Output voltage.
    Vout = 120;
    
    % Calculate load resistance assuming 100% efficiency.
    Rload = Vout^2 / P_assumed;
    % Transformer turns ratio.
    N = 1/5;
    % Effective AC resistance for voltage double rectifier converter.
    Rac = (8/pi^2) * (N^2) * (1/4) * Rload;
    
    % Define key parameters.
    K = Lm / Lr;
    Q = sqrt(Lr / Cr) / Rac;
    
    % Cubic equation's coefficients.
    a = 1;
    b = ((K^(-2)*(K+1)^2) - (2*Q^2) - (Gain^(-2))) / (Q^2);
    c = (Q^2 - (2*K^(-2) * (K + 1))) / (Q^2);
    d = (1 / (K * Q))^2;
    
    % Solve the cubic equation and take the square roots of the roots.
    fn_array = sqrt(roots([a b c d]));
    fn = max(real(fn_array));
    
    % Calculate resonance frequency.
    fr = 1 / (2 * pi * sqrt(Lr * Cr));
    
    % Estimated switching frequency.
    f0 = fn * fr;
end


function fsw = sliding_surface_control(Vref, Vpv, fold)
    % Define the sliding surface as the error between measured and desired output voltage.
    s = Vpv - Vref;

    % % Gain for sliding control (tune this value as needed).
    k_sliding = 2.0e3;  
    % Adaptive gain based on error magnitude
    if abs(s) < 2
        k_sliding = 1e3;
    elseif abs(s) < 4
        k_sliding = 3e3;
    elseif abs(s) < 6
        k_sliding = 5e3;
    else
        k_sliding = 7e3;
    end

    % Define boundary layer for chattering reduction.
    epsilon = 2.1;

    % Sliding method.
    sat_s = s / (epsilon + abs(s));
    
    % Adjust the nominal switching frequency.
    fsw = fold - k_sliding * sat_s;
end


function [Vout_denorm, Pout_denorm, VGMPPT, PGMPPT] = tflite_predict(I1, I2, I3, Voc_M)
    net = loadTFLiteModel('CNN.tflite');
    % net = loadTFLiteModel('ANN.tflite');
    
    I = [I1 I2 I3];

    % Model mean and std values.
    mean_val = net.Mean;
    std_dev_val = net.StandardDeviation;
    
    % Constants of PV panel used.
    offset = 2.54;
    Voc = Voc_M + offset;
    T = 25 + (Voc - 12.64 * 3) / (-0.36099/100 * 12.64 * 3);
    Isc = 8.62 + (T - 25) * (0.06371/100*8.62);
    % Ptmp = [243.9714245, 217.0348, 189.4542];
    Pmax = 249.8472 + (T - 25) * (-0.4417/100*249.8472);

    % Normalize Inputs
    I_norm = I / Isc; 

    % Ensure correct type.
    x = double(I_norm');

    % Ensure row vector format.
    x = reshape(x, [3, 1]);  
    x = std_dev_val*x + mean_val;
    
    % Prediction.
    val = predict(net, x);
    
    % Denormalize outputs.
    Pout_norm = val(1:3);
    Vout_norm = val(4:6);
    
    % Normalize output.
    Pout_denorm = reshape(double(Pout_norm * Pmax), 1, []);  % Ensure [1x3]
    Vout_denorm = reshape(double(Vout_norm * Voc), 1, []);   % Ensure [1x3]

    

    % /////////////////////////////////////
    [PGMPPT, Index] = max(Pout_denorm);
    VGMPPT = Vout_denorm(Index);
end
